simulink model "chaine_base"  (R2023b)
settings: Solver=FixedStepDiscrete  StartTime=0.0  StopTime=Tsim  FixedStep=Te  RelTol=1e-3
values from neighbouring files (symbols this model uses):
  A = P.A    [parametres.m]    (also in parametres_chaine.m; partie3_q4.m; partie3_q5.m; partie3_q8.m = 1)
  d_ech = 1    [parametres_chaine.m]    (also in partie3_q12.m = d)
  graine = 1    [extension_source_huffman.m]    (also in mes_parametres.m = mod(sum(c .* (1:numel(c)) * 31) + 7 * numel(c), 2^31 - 1); parametres_chaine.m = P.graine; parametres_perso.m = mod(sum(c .* (1:numel(c)) * 31) + 7 * numel(c), 2^31 - 1); partie4_q10.m = P.graine)
  L = cell(0, 2)    [construire_chaine_qpsk.m]    (also in construire_chaine_qpsk_codee.m; construire_chaine_texte.m; construire_decodeur_hamming.m = {'Mot recu/1', 'Bits r/1'; parametres.m = P.L)
  p1 = P.p1    [parametres.m]    (also in parametres_chaine.m = 0.5; partie3_q4.m; partie3_q5.m; partie3_q8.m = 0.3)
  seuil = 0    [parametres_chaine.m]    (also in partie4_q10.m)
  sigma2 = N0 * L / (2 * Tb)    [parametres_chaine.m]    (also in partie3_q12.m; partie4_q10.m)
  Tb = 1    [parametres.m]    (also in parametres_chaine.m; partie3_simulation.m; partie4_q10.m = 7; partie5_q2.m)
  Te = Tb / L    [parametres.m]    (also in parametres_chaine.m; partie3_simulation.m)
libraries: simulink x3
settings Model: Creator=e2604176  LastModifiedBy=e2604176

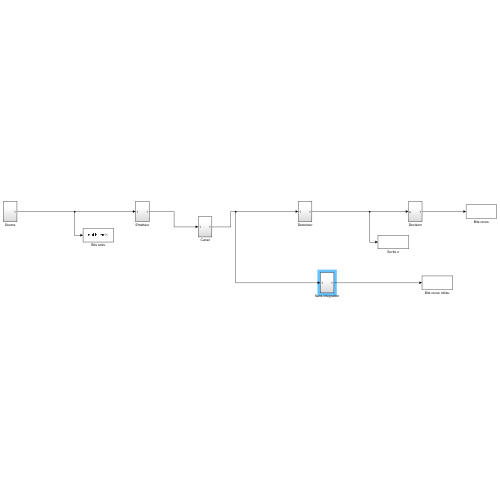
[thumbnail: Simulink's stored preview of the top-level diagram]
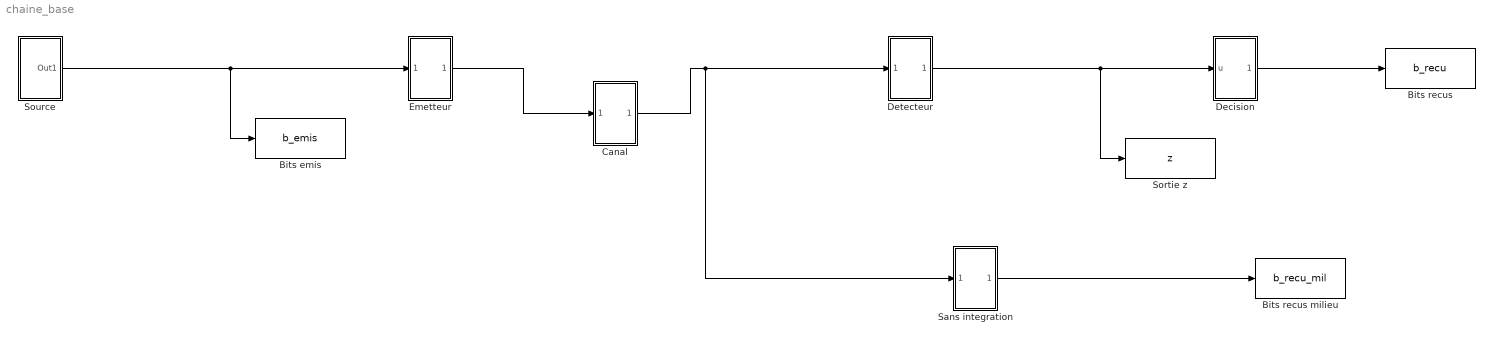
== system chaine_base ==
  Bits emis : ToWorkspace  VariableName=b_emis  SampleTime=-1
  Bits recus : ToWorkspace  VariableName=b_recu  SampleTime=-1
  Bits recus milieu : ToWorkspace  VariableName=b_recu_mil  SampleTime=-1
  Canal : Subsystem
  Decision : Subsystem
  Detecteur : Subsystem
  Emetteur : Subsystem
  Sans integration : Subsystem
  Sortie z : ToWorkspace  VariableName=z  SampleTime=-1
  Source : Subsystem
  wires:
  Source/1(Out1) -> Emetteur/1(In1), Bits emis/1
  Canal/1(Out1) -> Sans integration/1(In1), Detecteur/1(In1)
  Emetteur/1(Out1) -> Canal/1(In1)
  Detecteur/1(Out1) -> Decision/1(u), Sortie z/1
  Decision/1(Out1) -> Bits recus/1
  Sans integration/1(Out1) -> Bits recus milieu/1

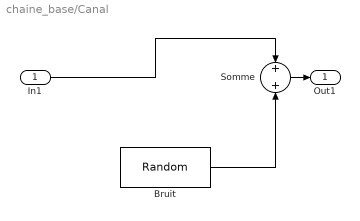
== system chaine_base/Canal ==
  In1 : Inport
  Bruit : RandomNumber  Variance=sigma2  Seed=graine + 1  SampleTime=Te
  Somme : Sum
  Out1 : Outport
  wires:
  Bruit/1 -> Somme/2
  Somme/1 -> Out1/1
  In1/1 -> Somme/1

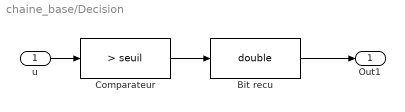
== system chaine_base/Decision ==
  u : Inport
  Bit recu : DataTypeConversion  OutDataTypeStr=double  SaturateOnIntegerOverflow=off  RndMeth=Floor
  Comparateur : simulink/Logic and Bit Operations/Compare To Constant  relop=>  const=seuil  OutDataTypeStr=boolean
  Out1 : Outport
  wires:
  u/1 -> Comparateur/1
  Comparateur/1 -> Bit recu/1
  Bit recu/1 -> Out1/1

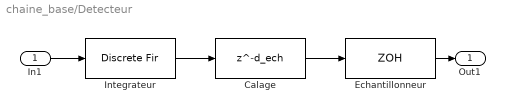
== system chaine_base/Detecteur ==
  In1 : Inport
  Calage : Delay  DelayLength=d_ech
  Echantillonneur : ZeroOrderHold  SampleTime=Tb
  Integrateur : DiscreteFir  Coefficients=ones(1, L) / L  SampleTime=Te
  Out1 : Outport
  wires:
  Echantillonneur/1 -> Out1/1
  Calage/1 -> Echantillonneur/1
  Integrateur/1 -> Calage/1
  In1/1 -> Integrateur/1

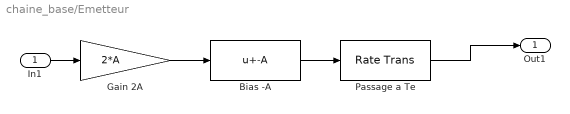
== system chaine_base/Emetteur ==
  In1 : Inport
  Bias -A : Bias  Bias=-A  SaturateOnIntegerOverflow=off
  Gain 2A : Gain  Gain=2*A
  Passage a Te : RateTransition  OutPortSampleTime=Te
  Out1 : Outport
  wires:
  In1/1 -> Gain 2A/1
  Gain 2A/1 -> Bias -A/1
  Bias -A/1 -> Passage a Te/1
  Passage a Te/1 -> Out1/1

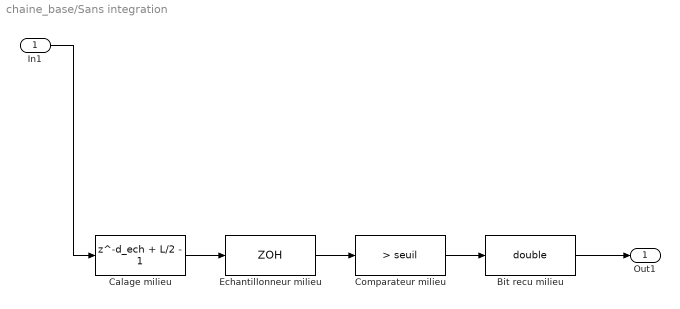
== system chaine_base/Sans integration ==
  In1 : Inport
  Bit recu milieu : DataTypeConversion  OutDataTypeStr=double  SaturateOnIntegerOverflow=off  RndMeth=Floor
  Calage milieu : Delay  DelayLength=d_ech + L/2 - 1
  Comparateur milieu : simulink/Logic and Bit Operations/Compare To Constant  relop=>  const=seuil  OutDataTypeStr=boolean
  Echantillonneur milieu : ZeroOrderHold  SampleTime=Tb
  Out1 : Outport
  wires:
  Calage milieu/1 -> Echantillonneur milieu/1
  Echantillonneur milieu/1 -> Comparateur milieu/1
  Comparateur milieu/1 -> Bit recu milieu/1
  Bit recu milieu/1 -> Out1/1
  In1/1 -> Calage milieu/1

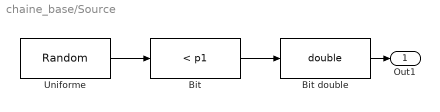
== system chaine_base/Source ==
  Bit : simulink/Logic and Bit Operations/Compare To Constant  relop=<  const=p1  OutDataTypeStr=boolean
  Bit double : DataTypeConversion  OutDataTypeStr=double  SaturateOnIntegerOverflow=off  RndMeth=Floor
  Uniforme : UniformRandomNumber  Minimum=0  Seed=graine  SampleTime=Tb
  Out1 : Outport
  wires:
  Uniforme/1 -> Bit/1
  Bit/1 -> Bit double/1
  Bit double/1 -> Out1/1
